simulink model "FAST_11To14_MPC_beta"  (R2019a)
settings: Solver=FixedStepAuto  StartTime=0.0  StopTime=200  FixedStep=DT  RelTol=1e-3
values from neighbouring files (symbols this model uses):
  Cq = 0.0 0.0 0.0 0.0 0.0 0.0 0.0 0.0 0.0 0.0 0.0 0.0 0.0 0.0 0.0 0.0 0.0 0.0 0.0 0.0 0.0 0.0 0.0 0.0 0.0 0.0 0.0 0.0 0.0 0.0 0.0 0.0 0.0 0.0 0.0 0.0 0.0 0.0 0.0 0.0 0.0 0.0 0.0 0.0 0.0 0.0 0.0 0.0 0.0 0.0 0.0 0.0 0.0 0.0 0.0 0.0 0.0 0.0 0.0 0.0 0.0 0.0 0.0 0.0 0.0 0.0 0.0 0.0 0.0 0.0 0.0 0.0 0.0 0.0 0.0 0.0 0.0 0.0 0.0 0.0 0.0 0.0 0.0 0.0 0.0 0.0 0.0 0.0 0.0 0.0 0.0 0.0 0.0 0.0 0.0 0.0 0.0 0.0 0.0 0.0    [DD_test.sldd]    (also in testOutList.m = saveVarsMat.Cq)
  Drivetrain = struct    [dataDLR.m]
  DT = 0.008    [dataDLR.m]    (also in generateReport.m; initLPVParam.m; initWorkspace.m; runCalculateEvalCriteria.m)
  Lin_points : value not decoded    [DD_test.sldd]
  mu_old = zeros(2*N*nu,1)    [testCtrl.m]
  Ng = 97    [dataDLR.m]    (also in testCtrl.m)
  omegabar = interp1(Lin_points.V,Lin_points.RSpeed,Vbar,'spline')    [testCtrl.m]
  OutList = OutTable.Properties.VariableNames    [initLPVParam.m]    (also in testCtrl.m; testOutList.m = cell(40, 1); testqLPV.m = cell(40, 1))
  U = zeros(2*N,1)    [testCtrl.m]
  Xk07 = kron(ones(N,1),xk07)    [testCtrl.m]
  xk07 = [r7(1), r7(2), zeros(1,5),0]'    [testCtrl.m]
undefined symbols (not defined in the file or in its folder): Rotor_Lambda, Rotor_Lamda, Rotor_Pitch, strmatch
libraries: MdlLib_ProcessOutput x1
settings Model: ExtModeTrigMode=oneshot  ExtModeArmWhenConnect=off  Creator=Hazim Namik  LastModifiedBy=ditt_aj
settings DataIOCC: LimitDataPoints=on  SaveFormat=Array  ReturnWorkspaceOutputs=off
settings OptimizationCC: BlockReduction=off  BooleanDataType=off  LifeSpan=inf
settings DebuggingCC: SaveWithParameterizedLinksMsg=none  UnderspecifiedInitializationDetection=Classic  MergeDetectMultiDrivingBlocksExec=none  SignalResolutionControl=TryResolveAllWithWarning  SFUnexpectedBacktrackingDiag=warning  SFNoUnconditionalDefaultTransitionDiag=warning  SFExecutionAtInitializationDiag=none  ArithmeticOperatorsInVariantConditions=warning
settings HardwareCC: ProdBitPerPointer=32  ProdBitPerSizeT=32  ProdBitPerPtrDiffT=32  ProdLargestAtomicFloat=None  ProdIntDivRoundTo=Undefined  ProdEndianess=Unspecified  ProdWordSize=32  ProdHWDeviceType=32-bit Generic  TargetUnknown=on
settings ModelReferenceCC: PropagateSignalLabelsOutOfModel=off
settings SFSimCC: SimUseLocalCustomCode=off
settings RTWCC: RTWUseLocalCustomCode=off
settings CodeAppCC: StateflowObjectComments=on
settings GRTTargetCC: TargetLangStandard=C89/C90 (ANSI)  GeneratePreprocessorConditionals=Disable all
settings ConfigComp: CovMetricSettings=dw  CovHtmlReporting=on  CovSaveCumulativeToWorkspaceVar=on  CovSaveSingleToWorkspaceVar=on  CovExternalEMLEnable=off

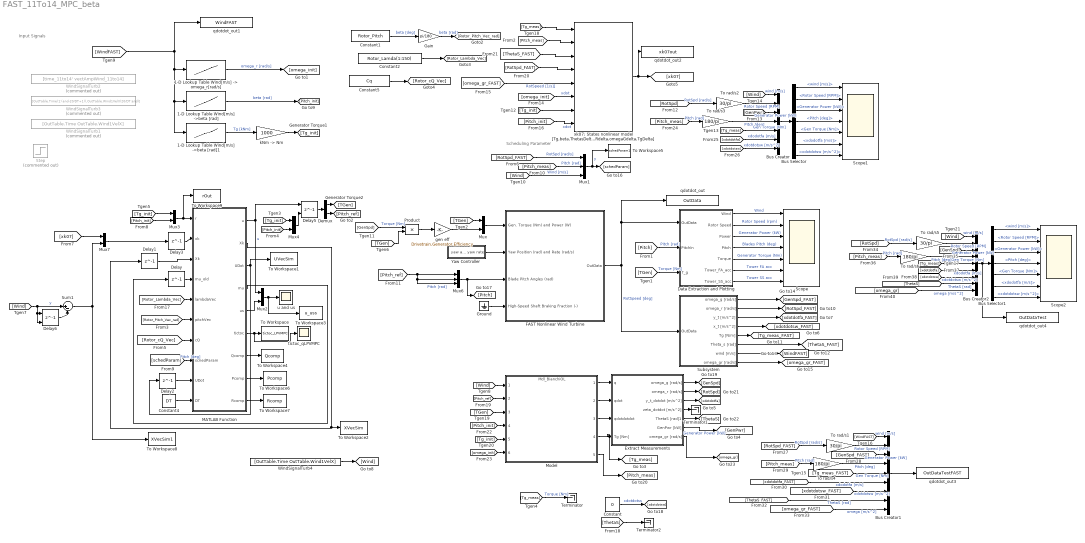
== system FAST_11To14_MPC_beta ==
  note: Input Signals
  note: Scheduling Parameter
  "1-D Lookup Table Wind[m/s] -> omega_r[rad/s]" : Lookup_n-D  NumberOfTableDimensions=1  BreakpointsForDimension1=Lin_points.V  BreakpointsForDimension2=Rotor_Lambda  Table=Lin_points.RSpeed  InternalRulePriority=Speed  RndMeth=Simplest  InputSameDT=on
  1-D Lookup Table Wind[m/s] ->beta [rad] : Lookup_n-D  NumberOfTableDimensions=1  BreakpointsForDimension1=Lin_points.V  BreakpointsForDimension2=Rotor_Lambda  Table=Lin_points.Pitch  InternalRulePriority=Speed  RndMeth=Simplest  InputSameDT=on
  1-D Lookup Table Wind[m/s] ->beta [rad]1 : Lookup_n-D  NumberOfTableDimensions=1  BreakpointsForDimension1=Lin_points.V  BreakpointsForDimension2=Rotor_Lambda  Table=Lin_points.Torque  InternalRulePriority=Speed  RndMeth=Simplest  InputSameDT=on
  Bus Creator : BusCreator  Inputs=7
  Bus Creator1 : BusCreator  Inputs=9
  Bus Creator2 : BusCreator  Inputs=9
  Bus Selector : BusSelector  OutputSignals=wind [m/s],Rotor Speed [RPM],Generator Power [kW],Pitch [deg],Gen Torque [Nm],xdodotfa [m/s],xdotdotsw [m/s^2]
  Bus Selector1 : BusSelector  OutputSignals=wind [m/s],Rotor Speed [RPM],Generator Power [kW],Pitch [deg],Gen Torque [Nm],xdodotfa [m/s],xdotdotsw [m/s^2]
  Constant : Constant  Value=0
  Constant1 : Constant  Value=Rotor_Pitch
  Constant2 : Constant  Value=Rotor_Lamda(1:150)
  Constant4 : Constant  Value=DT
  Constant5 : Constant  Value=Cq
  Data Extraction and Plotting : Subsystem
  Delay : Delay  DelayLength=1  InitialCondition=mu_old
  Delay1 : Delay  DelayLength=1  InitialCondition=Xk07
  Delay2 : Delay  DelayLength=1  InitialCondition=U
  Delay3 : Delay  DelayLength=1  InitialCondition=xk07
  Delay5 : Delay  DelayLength=1  InitialConditionSource=Input port  InitialCondition=[0,omegabar]
      settings: InputPortMap=u0,p4
  Delay6 : Delay  DelayLength=1  InitialConditionSource=Input port  InitialCondition=[0, Lin_points.Torque(1)]
      settings: InputPortMap=u0,p4
  Demux : Demux  Outputs=2
  Extract Measurements : Subsystem
  FAST Nonlinear Wind Turbine : Subsystem  mask(FAST Nonlinear Wind Turbine){}
      mask help: This block contains the FAST S-Function.
      mask init:
      | clear FAST_SFunc
  Gain : Gain  Gain=pi/180
  Ground : Ground
  MATLAB Function : MATLAB Function  TreatAsAtomicUnit=on
  Model : ModelReference  ModelNameDialog=Mdl_BianchiOL.slx  SimulationMode=Normal  ModelReferenceVersion=1.31
  Mux{,2..4,7} (5 alike) : Mux  Inputs=2
  Mux1 : Mux  Inputs=3
  Mux6 : Mux  Inputs=3
  Product : Product  RndMeth=Zero
  Scope : Scope  NumInputPorts=7
      settings: Tag=Scope
  Scope1 : Scope  NumInputPorts=7
      settings: Tag=Scope
  Scope2 : Scope  NumInputPorts=7
      settings: Tag=Scope
  Step : Step  Commented=on  Time=0  Before=9.9960  After=11  SampleTime=0
  Subsystem : Subsystem
  Sum1 : Sum  Inputs=|+-
  Terminator : Terminator
  Terminator1 : Terminator
  Terminator2 : Terminator
  To Workspace : ToWorkspace  VariableName=tictoc_LPVMPC  SaveFormat=Timeseries  SampleTime=-1
  To Workspace1 : ToWorkspace  VariableName=UVecSim  SampleTime=-1
  To Workspace2 : ToWorkspace  VariableName=XVecSim  SampleTime=-1
  To Workspace3 : ToWorkspace  VariableName=u_uss  SampleTime=-1
      settings: Save2DSignal=2-D array (concatenate along first dimension)
  To Workspace4 : ToWorkspace  VariableName=Qcomp  SampleTime=-1
      settings: Save2DSignal=2-D array (concatenate along first dimension)
  To Workspace5 : ToWorkspace  VariableName=schedParam1  SampleTime=-1
      settings: Save2DSignal=2-D array (concatenate along first dimension)
  To Workspace6 : ToWorkspace  VariableName=Pcomp  SampleTime=-1
      settings: Save2DSignal=2-D array (concatenate along first dimension)
  To Workspace7 : ToWorkspace  VariableName=Rcomp  SampleTime=-1
      settings: Save2DSignal=2-D array (concatenate along first dimension)
  To Workspace8 : ToWorkspace  VariableName=XVecSim1  SampleTime=-1
  To Workspace9 : ToWorkspace  VariableName=rOut  SampleTime=-1
  To rad/s1 : Gain  Gain=30/pi
  To rad/s2 : Gain  Gain=30/pi
  To rad/s3 : Gain  Gain=180/pi
  To rad/s4 : Gain  Gain=180/pi
  To rad/s5 : Gain  Gain=30/pi
  To rad/s6 : Gain  Gain=180/pi
  WindSignalTurb1 : FromWorkspace  Commented=on  VariableName=[OutTable.Time OutTable.Wind1VelX]  SampleTime=DT  OutputAfterFinalValue=Holding final value
  WindSignalTurb2 : FromWorkspace  Commented=on  VariableName=[time_11to14' vectAmpWind_11to14]  SampleTime=DT  OutputAfterFinalValue=Holding final value
  WindSignalTurb3 : FromWorkspace  Commented=on  VariableName=[OutTable.Time(1:(end-20/DT+1)),OutTable.Wind1VelX(20/DT:end)]  SampleTime=DT  OutputAfterFinalValue=Holding final value
  WindSignalTurb4 : FromWorkspace  VariableName=[OutTable.Time OutTable.Wind1VelX]  SampleTime=DT  OutputAfterFinalValue=Holding final value
  Yaw Controller : Subsystem
  gen eff : Gain  Gain=Drivetrain.Generator.Efficiency
  "kNm -> Nm" : Gain  Gain=1000
  qdotdot_out : ToWorkspace  VariableName=OutData  SampleTime=-1
  qdotdot_out1 : ToWorkspace  VariableName=WindFAST  SampleTime=-1
  qdotdot_out2 : ToWorkspace  VariableName=xk07out  SampleTime=-1
  qdotdot_out3 : ToWorkspace  VariableName=OutDataTestFAST  SampleTime=-1
  qdotdot_out4 : ToWorkspace  VariableName=OutDataTest  SampleTime=-1
  tictoc_qLPVMPC : Scope
  u and us : Scope
  xk07: States nonlinear model [Tg,beta,ThetasDelta,omegaRdelta,omegaGdelta,TgDelta] : MdlLib_ProcessOutput/xk07: States nonlinear model [Tg,beta,ThetasDelta,omegaRdelta,omegaGdelta,TgDelta]  SystemSampleTime=-1
  wires:
  Mux/1 -> FAST Nonlinear Wind Turbine/1(Gen. Torque (Nm) and Power (W))
  Yaw Controller/1(yaw and yaw rate) -> FAST Nonlinear Wind Turbine/2(Yaw Position (rad) and Rate (rad/s))
  gen eff/1 -> Mux/2
  Product/1 -> gen eff/1
  Data Extraction and Plotting/3(Power) -> Scope/3  "Generator Power (kW)"
  [Pitch] -> Data Extraction and Plotting/2(PitchIn)  "Pitch [rad]"
  Data Extraction and Plotting/1(Wind) -> Scope/1  "Wind"
  Data Extraction and Plotting/2(Rotor Speed) -> Scope/2  "Rotor Speed (rpm)"
  [TGen] -> Data Extraction and Plotting/3(T_g)  "Torque [Nm]"
  Data Extraction and Plotting/4(Pitch) -> Scope/4  "Blades Pitch (deg)"
  Data Extraction and Plotting/5(Torque) -> Scope/5  "Generator Torque (Nm)"
  Data Extraction and Plotting/6(Tower_FA_acc) -> Scope/6  "Tower FA acc"
  Data Extraction and Plotting/7(Tower_SS_acc) -> Scope/7  "Tower SS acc"
  Ground/1 -> FAST Nonlinear Wind Turbine/4(High-Speed Shaft Braking Fraction (-))
  [TGen] -> Mux/1
  Constant5/1 -> [Rotor_cQ_Vec]
  Gain/1 -> [Rotor_Pitch_Vec_rad]  "beta [rad]"
  "1-D Lookup Table Wind[m/s] -> omega_r[rad/s]"/1 -> [omega_init]  "omega_r [rad/s]"
  Constant1/1 -> Gain/1  "beta [deg]"
  1-D Lookup Table Wind[m/s] ->beta [rad]/1 -> [Pitch_init]  "beta [rad]"
  [WindFAST] -> "1-D Lookup Table Wind[m/s] -> omega_r[rad/s]"/1, 1-D Lookup Table Wind[m/s] ->beta [rad]/1, 1-D Lookup Table Wind[m/s] ->beta [rad]1/1, qdotdot_out1/1
  1-D Lookup Table Wind[m/s] ->beta [rad]1/1 -> "kNm -> Nm"/1  "Tg [kNm]"
  "kNm -> Nm"/1 -> [Tg_init]
  Constant2/1 -> [Rotor_Lambda_Vec]
  FAST Nonlinear Wind Turbine/1(OutData) -> Subsystem/1(OutData), Data Extraction and Plotting/1(OutData), qdotdot_out/1  "RotSpeed [deg]"
  [Pitch_ref] -> Mux6/1, Mux6/3, Mux6/2  "Pitch [rad]"
  Mux6/1 -> [Pitch], FAST Nonlinear Wind Turbine/3(Blade Pitch Angles (rad))
  [TGen] -> Product/2
  [GenSpd] -> Product/1  "Torque [Nm]"
  Subsystem/5(Tg [N/m]) -> [Tg_meas_FAST]
  Subsystem/1(omega_g [rad/s]) -> [GenSpd_FAST]
  Subsystem/7(wind [m/s]) -> [WindFAST]
  Subsystem/6(Theta_s [rad]) -> [ThetaS_FAST]
  Subsystem/8(omega_gr [rad/s]) -> [omega_gr_FAST]
  Subsystem/3(y_t [m/s^2]) -> [xdotdotfa_FAST]
  Subsystem/2(omega_r [rad/s]) -> [RotSpd_FAST]
  Subsystem/4(x_t [m/s^2]) -> [xdotdotsw_FAST]
  [Tg_meas] -> Terminator/1  "Torque [Nm]"
  [Pitch_meas] -> Mux1/2  "Pitch [rad]"
  Mux1/1 -> To Workspace5/1, [schedParam]  "y"
  [RotSpd_FAST] -> Mux1/1  "RotSpd [rad/s]"
  [Wind] -> Mux1/3  "Wind [m/s]"
  [ThetaS_FAST] -> xk07: States nonlinear model [Tg,beta,ThetasDelta,omegaRdelta,omegaGdelta,TgDelta]/3
  [Tg_meas] -> xk07: States nonlinear model [Tg,beta,ThetasDelta,omegaRdelta,omegaGdelta,TgDelta]/1
  [Pitch_init] -> xk07: States nonlinear model [Tg,beta,ThetasDelta,omegaRdelta,omegaGdelta,TgDelta]/8  "xdot"
  [Tg_init] -> xk07: States nonlinear model [Tg,beta,ThetasDelta,omegaRdelta,omegaGdelta,TgDelta]/7
  [omega_init] -> xk07: States nonlinear model [Tg,beta,ThetasDelta,omegaRdelta,omegaGdelta,TgDelta]/6  "xdot"
  [RotSpd_FAST] -> xk07: States nonlinear model [Tg,beta,ThetasDelta,omegaRdelta,omegaGdelta,TgDelta]/4
  xk07: States nonlinear model [Tg,beta,ThetasDelta,omegaRdelta,omegaGdelta,TgDelta]/1 -> qdotdot_out2/1, [xk07]
  [Pitch_meas] -> xk07: States nonlinear model [Tg,beta,ThetasDelta,omegaRdelta,omegaGdelta,TgDelta]/2
  [omega_gr_FAST] -> xk07: States nonlinear model [Tg,beta,ThetasDelta,omegaRdelta,omegaGdelta,TgDelta]/5  "RotSpeed [1/s]]"
  MATLAB Function/3(UDot) -> Delay2/1, To Workspace1/1
  Constant4/1 -> MATLAB Function/10(DT)
  [Tg_init] -> Mux3/1
  Delay2/1 -> MATLAB Function/9("UDot ")
  Delay6/1 -> Sum1/2
  Demux/1 -> [TGen]
  MATLAB Function/7(Qcomp) -> To Workspace4/1
  [Rotor_cQ_Vec] -> MATLAB Function/7(cQ)
  [xk07] -> Mux7/1
  Demux/2 -> [Pitch_ref]
  Mux7/1 -> Delay3/1
  [Pitch_init] -> Mux4/2
  Mux4/1 -> Delay5/2
  Delay3/1 -> MATLAB Function/2(xk)
  [Wind] -> Delay6/2, Delay6/1, Sum1/1  "y"
  Delay5/1 -> Demux/1
  MATLAB Function/4(mu) -> Delay/1
  MATLAB Function/1(u) -> Delay5/1, Mux2/1  "u"
  Delay/1 -> MATLAB Function/4(mu_old)
  [Tg_init] -> Mux4/1
  MATLAB Function/2(Xk) -> Delay1/1, To Workspace2/1
  MATLAB Function/5(us) -> Mux2/2
  MATLAB Function/6(tictoc) -> tictoc_qLPVMPC/1, To Workspace/1
  Delay1/1 -> MATLAB Function/3("Xk ")
  Sum1/1 -> To Workspace8/1, Mux7/2
  MATLAB Function/9(Rcomp) -> To Workspace7/1
  [Rotor_Pitch_Vec_rad] -> MATLAB Function/6(pitchVec)
  Mux3/1 -> To Workspace9/1, MATLAB Function/1(r)
  Mux2/1 -> u and us/1, To Workspace3/1
  [schedParam] -> MATLAB Function/8(schedParam)  "Pitch [deg]"
  MATLAB Function/8(Pcomp) -> To Workspace6/1
  [Pitch_init] -> Mux3/2
  [Rotor_Lambda_Vec] -> MATLAB Function/5(lambdaVec)
  [omega_init] -> Model/6
  Model/5 -> [Pitch_meas]
  Extract Measurements/4(zeta_dotdot [m/s^2]) -> Terminator1/1
  Extract Measurements/2(omega_r [rad/s]) -> [RotSpd]
  [Pitch_init] -> Model/4
  Extract Measurements/6(GenPwr [kW]) -> [GenPwr]  "Generator Power [kW]"
  Model/2 -> Extract Measurements/2(qdot)
  [Tg_init] -> Model/5
  Model/3 -> Extract Measurements/3(qdotdotdot)
  Model/1 -> Extract Measurements/1(q)
  Extract Measurements/1(omega_g [rad/s]) -> [GenSpd]
  Model/4 -> [Tg_meas], Extract Measurements/4(Tg [Nm])
  Extract Measurements/5(ThetaS [rad]1) -> [ThetaS]
  [Pitch_ref] -> Model/2
  Extract Measurements/3(y_t_dotdot [m/s^2]) -> [xdotdotfa]
  [TGen] -> Model/3
  [Wind] -> Model/1
  Constant/1 -> [xdotdotsw]  "xdotdotss"
  [ThetaS] -> Terminator2/1
  Extract Measurements/7(omega_gr [rad/s]) -> [omega_gr]
  Bus Selector/1 -> Scope1/1  "<wind [m/s]>"
  Bus Selector/7 -> Scope1/7  "<xdotdotsw [m/s^2]>"
  Bus Selector/2 -> Scope1/2  "<Rotor Speed [RPM]>"
  [RotSpd] -> To rad/s2/1  "RotSpd [rad/s]"
  Bus Selector/3 -> Scope1/3  "<Generator Power [kW]>"
  Bus Selector/5 -> Scope1/5  "<Gen Torque [Nm]>"
  [xdotdotfa] -> Bus Creator/6  "xdodotfa [m/s]"
  To rad/s3/1 -> Bus Creator/4  "Pitch [deg]"
  To rad/s2/1 -> Bus Creator/2  "Rotor Speed [RPM]"
  Bus Selector/4 -> Scope1/4  "<Pitch [deg]>"
  [Wind] -> Bus Creator/1  "wind [m/s]"
  Bus Selector/6 -> Scope1/6  "<xdodotfa [m/s]>"
  [xdotdotsw] -> Bus Creator/7  "xdotdotsw [m/s^2]"
  [Tg_meas] -> Bus Creator/5  "Gen Torque [Nm]"
  [GenPwr] -> Bus Creator/3  "Generator Power [kW]"
  [Pitch_meas] -> To rad/s3/1  "Pitch [rad]"
  Bus Creator/1 -> Bus Selector/1
  [RotSpd_FAST] -> To rad/s1/1  "RotSpd [rad/s]"
  [WindFAST] -> Bus Creator1/1  "wind [m/s]"
  To rad/s4/1 -> Bus Creator1/4  "Pitch [deg]"
  [xdotdotfa_FAST] -> Bus Creator1/6  "xdodotfa [m/s]"
  To rad/s1/1 -> Bus Creator1/2  "Rotor Speed [RPM]"
  [xdotdotsw_FAST] -> Bus Creator1/7  "xdotdotsw [m/s^2]"
  [Pitch_meas] -> To rad/s4/1  "Pitch [rad]"
  Bus Creator1/1 -> qdotdot_out3/1
  [Tg_meas_FAST] -> Bus Creator1/5  "Gen Torque [Nm]"
  [GenSpd_FAST] -> Bus Creator1/3  "Generator Power [kW]"
  [ThetaS_FAST] -> Bus Creator1/8  "ThetaS [rad]"
  [omega_gr_FAST] -> Bus Creator1/9  "omega [m/s^2]"
  Bus Selector1/3 -> Scope2/3  "<Generator Power [kW]>"
  [RotSpd] -> To rad/s5/1  "RotSpd [rad/s]"
  [xdotdotsw] -> Bus Creator2/7  "xdotdotsw [m/s^2]"
  Bus Selector1/4 -> Scope2/4  "<Pitch [deg]>"
  To rad/s5/1 -> Bus Creator2/2  "Rotor Speed [RPM]"
  [Wind] -> Bus Creator2/1  "wind [m/s]"
  Bus Selector1/5 -> Scope2/5  "<Gen Torque [Nm]>"
  Bus Selector1/6 -> Scope2/6  "<xdodotfa [m/s]>"
  Bus Creator2/1 -> Bus Selector1/1, qdotdot_out4/1
  [Tg_meas] -> Bus Creator2/5  "Gen Torque [Nm]"
  [Pitch_meas] -> To rad/s6/1  "Pitch [rad]"
  [GenSpd] -> Bus Creator2/3  "Generator Power [kW]"
  To rad/s6/1 -> Bus Creator2/4  "Pitch [deg]"
  Bus Selector1/2 -> Scope2/2  "<Rotor Speed [RPM]>"
  [xdotdotfa] -> Bus Creator2/6  "xdodotfa [m/s]"
  Bus Selector1/1 -> Scope2/1  "<wind [m/s]>"
  Bus Selector1/7 -> Scope2/7  "<xdotdotsw [m/s^2]>"
  [ThetaS] -> Bus Creator2/8  "ThetaS [rad]"
  [omega_gr] -> Bus Creator2/9  "omega [m/s^2]"
  WindSignalTurb4/1 -> [Wind]

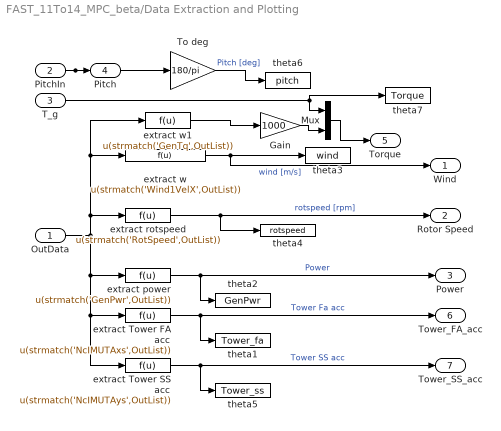
== system FAST_11To14_MPC_beta/Data Extraction and Plotting ==
  OutData : Inport
  PitchIn : Inport  Port=2
  T_g : Inport  Port=3
  Gain : Gain  Gain=1000
  Mux : Mux  Inputs=2
  To deg : Gain  Gain=180/pi
  extract Tower FA acc : Fcn  Expr=u(strmatch('NcIMUTAxs',OutList))
  extract Tower SS acc : Fcn  Expr=u(strmatch('NcIMUTAys',OutList))
  extract power : Fcn  Expr=u(strmatch('GenPwr',OutList))
  extract rotspeed : Fcn  Expr=u(strmatch('RotSpeed',OutList))
  extract w : Fcn  Expr=u(strmatch('Wind1VelX',OutList))
  extract w1 : Fcn  Expr=u(strmatch('GenTq',OutList))
  theta1 : ToWorkspace  VariableName=Tower_fa  SampleTime=-1
      settings: MaxDataPoints=Inf  Decimation=3
  theta2 : ToWorkspace  VariableName=GenPwr  SampleTime=-1
      settings: MaxDataPoints=Inf  Decimation=3
  theta3 : ToWorkspace  VariableName=wind  SampleTime=-1
      settings: MaxDataPoints=Inf  Decimation=3
  theta4 : ToWorkspace  VariableName=rotspeed  SampleTime=-1
      settings: MaxDataPoints=Inf  Decimation=3
  theta5 : ToWorkspace  VariableName=Tower_ss  SampleTime=-1
      settings: MaxDataPoints=Inf  Decimation=3
  theta6 : ToWorkspace  VariableName=pitch  SampleTime=-1
      settings: MaxDataPoints=Inf  Decimation=3
  theta7 : ToWorkspace  VariableName=Torque  SampleTime=-1
      settings: MaxDataPoints=Inf  Decimation=3
  Wind : Outport
  Rotor Speed : Outport  Port=2
  Power : Outport  Port=3
  Pitch : Outport  Port=4
  Torque : Outport  Port=5
  Tower_FA_acc : Outport  Port=6
  Tower_SS_acc : Outport  Port=7
  wires:
  extract w/1 -> Wind/1, theta3/1  "wind [m/s]"
  extract rotspeed/1 -> theta4/1, Rotor Speed/1  "rotspeed [rpm]"
  extract power/1 -> theta2/1, Power/1  "Power"
  PitchIn/1 -> To deg/1, Pitch/1
  T_g/1 -> Mux/1, theta7/1
  extract Tower FA acc/1 -> theta1/1, Tower_FA_acc/1  "Tower Fa acc"
  OutData/1 -> extract w/1, extract w1/1, extract rotspeed/1, extract Tower SS acc/1, extract Tower FA acc/1, extract power/1
  extract Tower SS acc/1 -> theta5/1, Tower_SS_acc/1  "Tower SS acc"
  extract w1/1 -> Gain/1
  Gain/1 -> Mux/2
  Mux/1 -> Torque/1
  To deg/1 -> theta6/1  "Pitch [deg]"

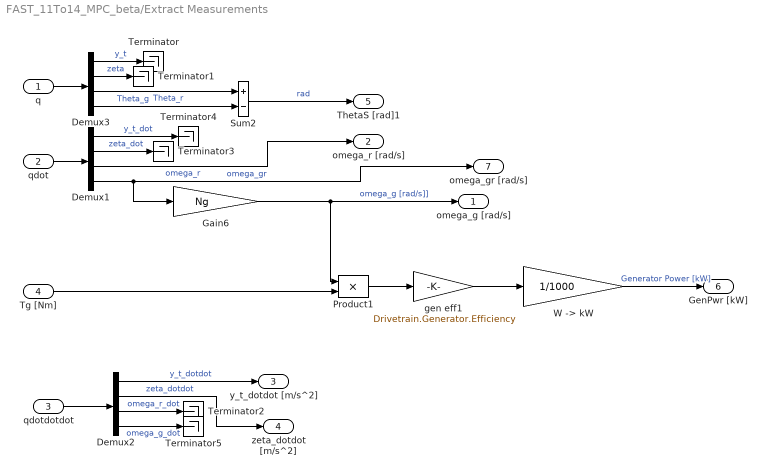
== system FAST_11To14_MPC_beta/Extract Measurements ==
  q : Inport
  qdot : Inport  Port=2
  qdotdotdot : Inport  Port=3
  Tg [Nm] : Inport  Port=4
  Demux1 : Demux
  Demux2 : Demux
  Demux3 : Demux
  Gain6 : Gain  Gain=Ng
  Product1 : Product  RndMeth=Zero
  Sum2 : Sum  Inputs=+-
  Terminator{,1..5} (6 alike) : Terminator
  "W -> kW" : Gain  Gain=1/1000
  gen eff1 : Gain  Gain=Drivetrain.Generator.Efficiency
  omega_g [rad/s] : Outport
  omega_r [rad/s] : Outport  Port=2
  y_t_dotdot [m/s^2] : Outport  Port=3
  zeta_dotdot [m/s^2] : Outport  Port=4
  ThetaS [rad]1 : Outport  Port=5
  GenPwr [kW] : Outport  Port=6
  omega_gr [rad/s] : Outport  Port=7
  wires:
  Demux1/2 -> Terminator3/1  "zeta_dot"
  Demux2/1 -> y_t_dotdot [m/s^2]/1  "y_t_dotdot"
  Gain6/1 -> Product1/1, omega_g [rad/s]/1  "omega_g [rad/s]]"
  Demux1/3 -> omega_r [rad/s]/1  "omega_r"
  Demux1/1 -> Terminator4/1  "y_t_dot"
  qdot/1 -> Demux1/1
  Demux3/3 -> Sum2/1  "Theta_r"
  Demux3/4 -> Sum2/2  "Theta_g"
  Demux2/4 -> Terminator5/1  "omega_g_dot"
  Tg [Nm]/1 -> Product1/2
  Demux2/3 -> Terminator2/1  "omega_r_dot"
  Sum2/1 -> ThetaS [rad]1/1  "rad"
  Demux1/4 -> omega_gr [rad/s]/1, Gain6/1  "omega_gr"
  Product1/1 -> gen eff1/1
  Demux3/2 -> Terminator1/1  "zeta"
  Demux2/2 -> zeta_dotdot [m/s^2]/1  "zeta_dotdot"
  Demux3/1 -> Terminator/1  "y_t"
  gen eff1/1 -> "W -> kW"/1
  "W -> kW"/1 -> GenPwr [kW]/1  "Generator Power [kW]"
  q/1 -> Demux3/1
  qdotdotdot/1 -> Demux2/1

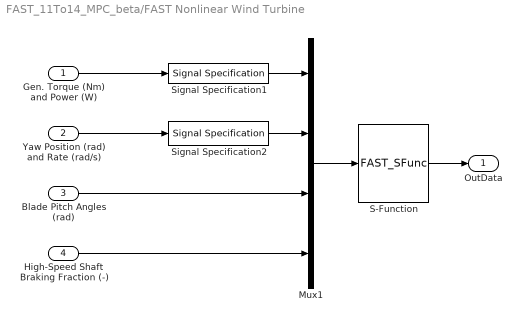
== system FAST_11To14_MPC_beta/FAST Nonlinear Wind Turbine ==
  Gen. Torque (Nm) and Power (W) : Inport
  Yaw Position (rad) and Rate (rad/s) : Inport  Port=2
  Blade Pitch Angles (rad) : Inport  Port=3
  High-Speed Shaft Braking Fraction (-) : Inport  Port=4
  Mux1 : Mux
  S-Function : S-Function  FunctionName=FAST_SFunc  Parameters=FAST_InputFileName, TMax, 0  SFunctionDeploymentMode=off  EnableBusSupport=off
  Signal Specification1 : SignalSpecification  OutDataTypeStr=double  Dimensions=2
  Signal Specification2 : SignalSpecification  OutDataTypeStr=double  Dimensions=2
  OutData : Outport
  wires:
  Gen. Torque (Nm) and Power (W)/1 -> Signal Specification1/1
  S-Function/1 -> OutData/1
  Mux1/1 -> S-Function/1
  Blade Pitch Angles (rad)/1 -> Mux1/3
  Yaw Position (rad) and Rate (rad/s)/1 -> Signal Specification2/1
  Signal Specification1/1 -> Mux1/1
  Signal Specification2/1 -> Mux1/2
  High-Speed Shaft Braking Fraction (-)/1 -> Mux1/4

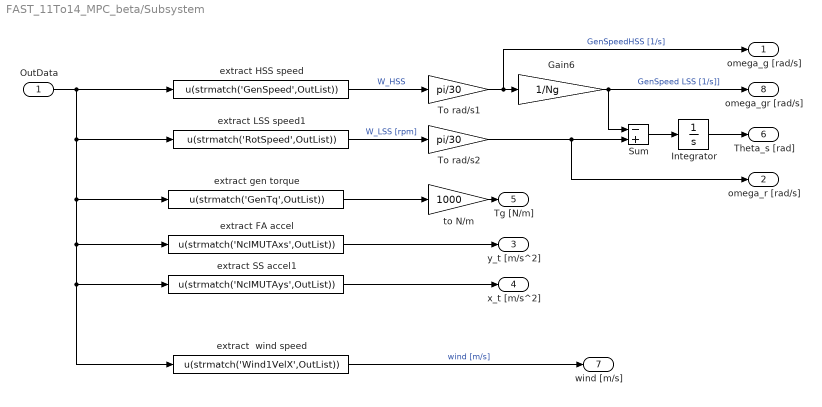
== system FAST_11To14_MPC_beta/Subsystem ==
  OutData : Inport
  Gain6 : Gain  Gain=1/Ng
  Integrator : Integrator
  Sum : Sum  Inputs=-+
  To rad/s1 : Gain  Gain=pi/30
  To rad/s2 : Gain  Gain=pi/30
  extract  wind speed : Fcn  Expr=u(strmatch('Wind1VelX',OutList))
  extract FA accel : Fcn  Expr=u(strmatch('NcIMUTAxs',OutList))
  extract HSS speed : Fcn  Expr=u(strmatch('GenSpeed',OutList))
  extract LSS speed1 : Fcn  Expr=u(strmatch('RotSpeed',OutList))
  extract SS accel1 : Fcn  Expr=u(strmatch('NcIMUTAys',OutList))
  extract gen torque : Fcn  Expr=u(strmatch('GenTq',OutList))
  to N/m : Gain  Gain=1000
  omega_g [rad/s] : Outport
  omega_r [rad/s] : Outport  Port=2
  y_t [m/s^2] : Outport  Port=3
  x_t [m/s^2] : Outport  Port=4
  Tg [N/m] : Outport  Port=5
  Theta_s [rad] : Outport  Port=6
  wind [m/s] : Outport  Port=7
  omega_gr [rad/s] : Outport  Port=8
  wires:
  to N/m/1 -> Tg [N/m]/1
  OutData/1 -> extract HSS speed/1, extract  wind speed/1, extract SS accel1/1, extract FA accel/1, extract gen torque/1, extract LSS speed1/1
  extract FA accel/1 -> y_t [m/s^2]/1
  extract HSS speed/1 -> To rad/s1/1  "W_HSS"
  extract gen torque/1 -> to N/m/1
  extract SS accel1/1 -> x_t [m/s^2]/1
  To rad/s1/1 -> omega_g [rad/s]/1, Gain6/1  "GenSpeedHSS [1/s]"
  extract LSS speed1/1 -> To rad/s2/1  "W_LSS [rpm]"
  Gain6/1 -> Sum/1, omega_gr [rad/s]/1  "GenSpeed LSS [1/s]]"
  To rad/s2/1 -> Sum/2, omega_r [rad/s]/1
  Sum/1 -> Integrator/1
  Integrator/1 -> Theta_s [rad]/1
  extract  wind speed/1 -> wind [m/s]/1  "wind [m/s]"

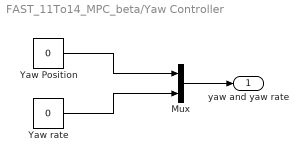
== system FAST_11To14_MPC_beta/Yaw Controller ==
  Mux : Mux  Inputs=2
  Yaw Position : Constant  Value=0
  Yaw rate : Constant  Value=0
  yaw and yaw rate : Outport
  wires:
  Mux/1 -> yaw and yaw rate/1
  Yaw Position/1 -> Mux/1
  Yaw rate/1 -> Mux/2

== matlab function FAST_11To14_MPC_beta/MATLAB Function ==
  settings: updateMethod=DISCRETE
  data: r input; u output; xk input; Xk input; mu_old input; lambdaVec input; pitchVec input; cQ input; schedParam input; UDot input; DT input; Xk output; UDot output; mu output; us output; tictoc output; Qcomp output; Pcomp output; Rcomp output
function [u,Xk,UDot,mu,us,tictoc, Qcomp,Pcomp,Rcomp]= qLPVMPC_WECS_beta(r,xk,Xk,mu_old,lambdaVec,pitchVec,cQ,schedParam,UDot,DT)
% MATLAB_Function calculates controller output u. It turns the QP into a 
% linear complementarity problem (LCP) and solves it with Lemke's algorithm.
%
% Inputs: * r: reference
%         * xk: quasiLPV KF state estimates
%         * Xk: Xko(= L*xk+S*U) delayed by one sample timestep
%         * mu_old: mu delayed by one sample timestep
%         * lambdaVec: lambda vector for cQ LUT 
%         * pitchVec: pitch vector for cQ LUT 
%         * cQ: torque coefficients LUT matrix
%         * schedParam: current values [omegaR, beta, V]
%         * U: U (from Xko = L*xk+S*U) delayed by one sample timestep
%
% Outputs: * u: controller output at current time step
%          * Xko: Future state trajectory (L*xk+S*U)
%          * U: Future input trajectory 
%          * mu: Result Lemke's algorithm/LCP: M mu +q >=0, mu>=0, mu'(Mmu+q)=0
%          * us: xuss(end) from xuss = [eye(4)-Ass -Bss;[1 0 0 0] 0]\[Bss*d;1]
%          * tictoc: tic-toc result

% Pablo S.G. Cisneros, Herbert Werner, ICS TUHH

%#codegen
coder.extrinsic('tic');
coder.extrinsic('toc');
tictoc = 0;
tic

%% Init N, Q, R
N = 40;
q_ = [1 10^3 0 10^3 10^3 0 0 0]; %[10^4 0.1 1 1 100 0.1 0]; %q_ = [100 1000 1 0.01 0]; 7.351e+02 1.000e+00 1.938e+09 1.625e+08 1.491e+08 1.657e+03
r_ = [1 10^4]; %[10^7,0.1];
R_ = kron(eye(N),diag(r_)); %R_ = 1000*eye(N); 
p = 10*q_; %P = 1000*diag(q_);

Ulim = repmat([20000,8 * pi/180]',2*N,1); %rate constraints 

Control_Pitch_Max = 90 /180 * pi;
Control_Pitch_Min = 0 /180 * pi;
Control_Torque_Limit = 47403;
Control_Torque_Min = 200;

% isBetaState = 0;
% nx = 4 + isBetaState; % number states plant: ThetaS,omegaR,omegaG,Tg
% ny = 2 + isBetaState; % number of outputs plant omegaG,Tg
nxA = 8;% nx + ny +clc 1; %number states augmented plant 
nu = 2; % plant inputs: Tg_ref, beta_ref

%% Shift Xk
Xk(1:end-nxA) = Xk(nxA+1:end); 
UDot(1:end-nu) = UDot(nu+1:end);
%Xk(1:nxA)

%% Calculate input u_dot_s = 0  and steady state x = r
us = [0;0]; %xuss(nxA+1:nxA+2); % xuss = [eye(size(Ass))-Ass -Bss;[1 0 0 0] 0] \ [Bss*d;reference];

iterations = 1; % omega_ref(Vest), Tg_ref(Vest)
refVec = zeros(nxA,1);
refVec(1:2) = r;
ref = repmat(refVec,N,1); %ref = kron(ones(N,1),[r; 0; 0; 0;0]);

for i = 1:iterations
    [L,S,H,g] = HSqLd_WT_beta(N,q_,R_,p,xk,Xk,DT,ref,us,lambdaVec,pitchVec,cQ,schedParam,UDot);
    
    %% %%%%%%Turn QP into LCP and solve it%%%%%%%%%
    Ac_ = [-eye(N*nu);eye(N*nu)];
    bc_ = - Ulim;
    Hi = eye(size(H,1))/H;
    M = Ac_*Hi*Ac_';
    q = -Ac_*Hi*g - bc_;
 
    mu = lemke(M,q,mu_old);
 
    UDot = Hi*(Ac_'*mu-g);
    UDot(isnan(UDot)) = 0;
    
    %% %%%%%%%%%%%%%%%%%%%%%%%%%%%%%%%%%%%%%%%%%%%%    
    Xk = L*xk+S*UDot;
end

u =  [ min(max(UDot(1) + Xk(1), Control_Torque_Min),Control_Torque_Limit),... % torque
min( max(UDot(2) + Xk(2), Control_Pitch_Min),Control_Pitch_Max)]'; % pitch

tictoc = toc;

% For debugging
%%%%%%%%%%% Compute Hessian H, derivative g = dJk/dUk %%
% min Jk(Uk) s.t. h1(Uk) = 0, h2(Uk) < 0, at current estimate xl
% <=> min( x'H(xl)x + g(xl)x s.t. dh1(xl)x+h1(xl)=0, dh2(xl)x+h2(xl)< 0
% with 
% Jk = (Lx+SUk-Xss)'Q(Lx+SUk-Xss) +(Uk-Uss)'R(Uk-Uss) + Psi
% dJk/dUk = 2S'Q (Lx+SUk-Xss) + 2R(Uk-Uss) 
diffX = Xk(1:(end - nxA)) - ref(1:(end -nxA));
diffXEnd = Xk((end - nxA +1):end) - ref((end - nxA +1):end);

% Q_ = kron(eye(N-1),diag(q_));
% Qcomp = diffX' * Q_ * diffX;
% Pcomp = diffXEnd' * diag(p)* diffXEnd;
% Rcomp = U' * R_ * U;

diffXMat = sum(reshape(diffX.^2, nxA, N-1),2);
UMat = sum(reshape(UDot.^2, 2, N),2);

Qcomp = diffXMat' .* q_;
Pcomp = (diffXEnd') .^2  .* p;
Rcomp = UMat' .* r_;
